simulink model "Porsche930Turbo_Model_V0"  (R2025b)
settings: Solver=ode3  StartTime=0.0  StopTime=1800  FixedStep=0.005  MaxStep=0.01  RelTol=1e-3
values from neighbouring files (symbols this model uses):
  a_front = (1 - CoG_front) * wb    (= 1.32912)    [Main.m]
  af = 1.77    [Main.m]
  bsfc = 395    [Main.m]
  cd = 0.39    [Main.m]
  crr = 0.015    [Main.m]
  distance_imola = s_track    [Main.m]
  eta_gb = 0.95    [Main.m]
  gear_numbers = [1, 2, 3, 4]    [Main.m]
  gear_ratios = [2.25, 1.30, 0.89, 0.625]    [Main.m]
  gear_shift_tbl = [1, 2, 3, 4]    [Main.m]
  grade_imola = grade_track    [Main.m]
  kt = 1.65    [Main.m]
  m_eq = mg + (J_wheels / rw^2) + (J_drivetrain * i_avg^2 / rw^2)    [Main.m]
  mg = mc + (mh * np) + mp_hybrid    (= 1492.5)    [Main.m]
  mu_road = 0.9    [Main.m]
  n_ice = 0:dn:nd    [Main.m]
  ne_em = 0:dn:nemax_em    [Main.m]
  nparallel = 2    [Main.m]
  nseries = 96    [Main.m]
  rho_fuel = 0.75    [Main.m]
  ro = 1.204    [Main.m]
  rt = 4.222    [Main.m]
  rw = (dw * 25.4 / 2 + wt * art / 100) * 1e-3    (= 0.31345)    [Main.m]
  t_ice = zeros(size(n_ice))    [Main.m]
  t_roma_san_basilio = [0 1 2 3 4 5 6 7 8 9 10 11 ... (522 elements, 522x1)]    [ECE_EUDC_Artemis_Bologna_Roma_WLTC_EE_bus.mat]
  tau_turbo = 0.6    [Main.m]
  te_em = zeros(size(ne_em))    [Main.m]
  te_em_peak = zeros(size(ne_em))    [Main.m]
  temax_em = 230    [Main.m]
  tmax_ice = 412    [Main.m]
  track_length = 4909    [Main.m]
  v_cutoff_bp = [0, 0.5, 1.4, 50]    [Main.m]
  v_cutoff_tbl = [0, 0,   1,   1 ]    [Main.m]
  v_ref_imola = v_track_ms    [Main.m]
  v_shift_bp = [0, 18, 33, 48]    [Main.m]
  v_shift_bp_EMODE = [0, 5, 22, 35]    [Main.m]
  vkm_roma_san_basilio = [28.8 30.9 32.4 34.2 35.3 35.6 34.8 33.8 32.2 30.5 29.1 27.9 ... (522 elements, 522x1)]    [ECE_EUDC_Artemis_Bologna_Roma_WLTC_EE_bus.mat]
  wb = 2.272    [Main.m]
undefined symbols (not defined in the file or in its folder): SoC_Per
libraries: simulink x58
(part 5 of 5)

== system Porsche930Turbo_Model_V0/E-MOTOR/EM_model_v47b/Motor_Model/blockD/idq_max_MTC-I0/iq_mtcMax/0ck1 ==
  i : Inport
  Abs1 : Abs  SaturateOnIntegerOverflow=off
  Constant3 : Constant  Value=0
  Manual Switch3 : ManualSwitch  CurrentSetting=0
  MinMax1 : MinMax  Function=max  Inputs=2
  o : Outport
  wires:
  i/1 -> MinMax1/1, Abs1/1
  Abs1/1 -> Manual Switch3/1
  Manual Switch3/1 -> o/1
  MinMax1/1 -> Manual Switch3/2
  Constant3/1 -> MinMax1/2

== matlab function Porsche930Turbo_Model_V0/ECU/Hybrid_Mode/MATLAB Function ==
  settings: updateMethod=DISCRETE  sampleTime=0.01
  data: t_req input; t_ICE output; t_em output; t_em_max input; SoC input
function [t_ICE, t_em] = Engine_sweetspot_operation(t_req, t_em_max, SoC)

    %ENFORCE UNIFORM DOUBLE PRECISION (Prevents Coder Type-Mismatch)
    t_req    = double(t_req);
    t_em_max = double(t_em_max);
    SoC      = double(SoC);

    t_sweetspot = 380.0;   % [Nm] Optimal BSFC operating point (3.3L Boxer Turbo)

    % AUTOMATIC SOC NORMALIZATION
    if SoC > 1.0
        soc_norm = SoC / 100.0;
    else
        soc_norm = SoC;
    end

    % HIGH-SOC REGENERATION / RECHARGE DERATING (90% -> 95%)
    % Protects battery cells against overvoltage (4.2V/cell) and lithium plating.
    if soc_norm <= 0.90
        regen_factor = 1.0;
    elseif soc_norm < 0.95
        regen_factor = (0.95 - soc_norm) / 0.05;
    else
        regen_factor = 0.0; % Above 95%: Zero recharge allowed (t_em >= 0)
    end

    % HYSTERESIS RECOVERY STATE (20% -> 50%)
    persistent force_recharge;
    if isempty(force_recharge)
        force_recharge = false;
    end

    % Latch forced recharge below 20%, maintain until 50% is recovered
    if (soc_norm <= 0.20)
        force_recharge = true;
    elseif (soc_norm >= 0.50)
        force_recharge = false;
    end

    %TORQUE DISPATCHING (CONTINUOUS LAWS)
    if force_recharge
        %STATE A: FORCED BATTERY RECOVERY MODE
        if t_req <= 0.0
            % Deceleration / Braking: regenerative braking scaled by regen_factor
            t_ICE = 0.0;
            t_em  = regen_factor * max(t_req, -t_em_max);

        else
            % Smooth throttle tip-in charging ramp (0 to 80 Nm)
            % Eliminates the instant 230 Nm (45 kW) step jump on pedal touch
            k_ramp    = min(1.0, t_req / 80.0);
            t_gen_max = regen_factor * min(t_em_max, max(0.0, t_sweetspot - t_req));
            t_gen     = k_ramp * t_gen_max;

            t_ICE = t_req + t_gen;
            t_em  = -t_gen;
        end

    else
        % STATE B: NORMAL HYBRID MODE
        t_ev_max   = 90.0;    % [Nm] Pure EV threshold
        t_ice_full = 125.0;   % [Nm] Full sweet-spot threshold

        if t_req <= 0.0
            % Deceleration / Braking: scaled regenerative braking
            t_ICE = 0.0;
            t_em  = regen_factor * max(t_req, -t_em_max);

        elseif t_req <= t_ev_max
            % Low load: Pure Electric Vehicle (EV) mode
            t_ICE = 0.0;
            t_em  = t_req;

        elseif t_req < t_ice_full
            % Smooth linear blending zone (90 to 125 Nm)
            alpha          = (t_req - t_ev_max) / (t_ice_full - t_ev_max);
            t_charge_avail = regen_factor * t_em_max;
            t_target_ice   = min(t_sweetspot, t_req + t_charge_avail);
            
            t_ICE = alpha * t_target_ice;
            t_em  = t_req - t_ICE;

        elseif t_req <= t_sweetspot
            % Medium load: ICE sweet-spot charging modulated by regen_factor
            t_charge_avail = regen_factor * min(t_em_max, t_sweetspot - t_req);
            t_ICE = t_req + t_charge_avail;
            t_em  = -t_charge_avail;

        elseif t_req <= (t_sweetspot + t_em_max)
            % High load: ICE at 380 Nm + Electric Motor Boost assist
            t_ICE = t_sweetspot;
            t_em  = t_req - t_sweetspot;

        else
            % Peak load: Saturated electric boost + ICE
            t_em  = t_em_max;
            t_ICE = t_req - t_em;
        end
    end
end

== matlab function Porsche930Turbo_Model_V0/E-MOTOR/EM_model_v47b/Motor_Model/TF/ solver_TF ==
  data: a input; id output; iq output; discr output; r input; r1 input; b input; t input; theta input
function [id, iq, discr] = SolQuart_tf(a, r, r1, b, t, theta)
% [id, iq, discr] = SolQuart_tf(a, r, r1, b, t, theta)
% page 77 tesi liscio (torque follower with Ferrari's method)

thp2 = theta^2;
th1  = 1/thp2+1;
if r==1  %isomachine
    det = a^2-th1*(th1*t^2/a^2+2*t/theta+a^2-b^2);
    if det>=0
        id    = (-a+sqrt(det)) /th1;
        iq    = t/a;
        discr = 1;
    else
        id    = 0;
        iq    = 0;
        discr = 0;
    end
else    %every other case other than isomachine
    %r1 = 1-1/r;
    %risoluzione della quartica
    A1 = r^2*r1^2+r1^2/thp2;
    B1 = 2*a*r1^2*r^2+r^2*2*a*r1+2*a*r1/thp2;
    C1 = -2*t*r1/theta+2*r*t*r1/theta+a^2*r^2+a^2/thp2+r^2*a^2*r1^2+4*a^2*r^2*r1-b^2*r1^2;
    D1 = -2*t*a/theta+2*a*r*t/theta+2*a*r*t*r1/theta+2*a^3*r^2+2*r^2*a^3*r1-2*a*r1*b^2;
    E1 = th1*t^2+2*a^2*r*t/theta+r^2*a^4-b^2*a^2;

    A = B1/A1;
    B = C1/A1;
    C = D1/A1;
    D = E1/A1;

    Pr = A*C - 4*D - (B^2/3);
    Qr = 4*B*D -A^2*D - C^2+ B*(A*C-4*D)/3 - 2*(B^3/27);

    DeltaR = (Qr^2/4) + (Pr^3/27);
    
    if DeltaR>0 %studio il discriminante per vedere se è correlato alla id_TF
        Sdelt = sqrt(DeltaR);
        temp1 = -Qr/2+Sdelt;
        temp2 = -Qr/2-Sdelt;
        Ur  = sign(temp1) * (abs(temp1))^(1/3);
        Vr  = sign(temp2) * (abs(temp2))^(1/3);
        S1r = Ur+Vr+B/3;
    else
        thetag = atan(sqrt(-DeltaR)/(-Qr/2));
        if thetag<0
            thetag = thetag+pi;
        end
        S1r = 2*sqrt(-Pr/3)*cos((thetag)/3)+B/3;
    end
    
    temp1 = sqrt((A^2/4)-B+S1r);
    temp2 = (-C+A*S1r/2) / (2*(A^2/4-B+S1r));
    %soluzioni quartica (utili)(valide solo se discr>0)
    
    if r<1
        I   = (A/2)   + temp1;
        L   = (S1r/2) + temp1 * temp2;
        det = I^2-4*L;
        if det<0
            id = 0;
        else
            id = 0.5* (-I + sqrt(det));
        end
    else
        G   = (A/2)   - temp1;
        H   = (S1r/2) - temp1 * temp2;
        det = G^2-4*H;
        if det<0
            id = 0;
        else
            id = 0.5* (-G + sqrt(det));
        end
    end
    
    if id==0
        iq    = 0;
        discr = 0;
    else
        iq    = t/(a+r1*id);
        discr = 1;
    end
end

end %fcn end

== matlab function Porsche930Turbo_Model_V0/E-MOTOR/EM_model_v47b/Motor_Model/blockD/idq_max_MTV-I0/intersections_neg ==
  data: a input; id output; iq output; discr output; r input; b input; I0 input; theta input; t input
function[id, iq, discr] = SolQuart_tfrs(a, r, b, I0, theta, t)
% [id, iq, discr] = SolQuart_tfrs(a, r, b, I0, theta, t)

thp2 = theta^2;
th1  = 1/thp2+1;
if r==1   %isomachine
    At  = (+I0^2*th1*thp2/a+thp2*a-thp2*b^2/a);
    Bt  = -I0^2+I0^4*th1^2*thp2/4/a^2+a^2*thp2/4+b^4*thp2/4/a^2+I0^2*...
          th1*thp2/2-I0^2*th1*thp2/a^2*b^2/2-thp2*b^2/2;
    det = At^2-4*(1+thp2)*Bt;
    if det>=0
        if t>=0
            id = (-At -sqrt(det)) / (2*(1+thp2));
        else
            id = (-At +sqrt(det)) / (2*(1+thp2));
        end
        iq   = -I0^2*th1*theta/(2*a)-id*theta-a*theta/2+b^2*theta/(2*a);
        discr = 0;
    else
        id    = 1000;
        iq    = 0;
        discr = 1;
    end

else      %every other case other than isomachine
    % risoluzione quartica (a,b,c,d a pag. 75, eq 3.31 )
    A1 = -4/thp2-4*r^2/thp2+8*r/thp2-th1^2-r^4-1/theta^4+2*th1*r^2+2*th1/thp2-2*r^2/thp2;
    B1 = 8*a*r/thp2-8*a*r^2/thp2+4*th1*a*r^2-4*r^4*a-4/thp2*a*r^2;
    C1 = 4/thp2*I0^2+4*r^2/thp2*I0^2-8*r/thp2*I0^2- 4*a^2*r^2/thp2+2*...
         th1^2*I0^2-4*a^2*r^4-2*b^2*th1+2*b^2*r^2+2*b^2/thp2+2*th1*a^2*r^2-2*...
         th1*I0^2*r^2-2*th1*I0^2/thp2-2*a^2*r^2/thp2-2*a^2*r^4;
    D1 = -8*a*r/thp2*I0^2+8*a*r^2*I0^2/thp2+4*b^2*a*r^2-4*I0^2*th1*a*r^2-4*a^3*r^4;
    E1 = 4*a^2*r^2*I0^2/thp2-b^4-th1^2*I0^4-a^4*r^4+2*b^2*th1*I0^2+2*b^2*a^2*r^2-2*I0^2*a^2*r^2*th1;

    A = B1/A1;
    B = C1/A1;
    C = D1/A1;
    D = E1/A1;
    
    Pr = A*C - 4*D - (B^2/3);
    Qr = 4*B*D - A^2*D - C^2 + B*(A*C-4*D)/3 - 2*(B^3/27);
    
    DeltaR = (Qr^2/4) + (Pr^3/27);
    
    if DeltaR>=0 
        %(se il discriminante è >0, allora il radicando è reale. Facendo la radice
        %cubica si ottiene una soluzione reale e 2 immaginarie. Le immaginarie
        %si ottengono moltiplicando la reale per (-1/2 +- irad3/2).
        Sdelt = sqrt(DeltaR);
        temp1 = -Qr/2+Sdelt;
        temp2 = -Qr/2-Sdelt;
        Ur  = sign(temp1) * (abs(temp1))^(1/3);
        Vr  = sign(temp2) * (abs(temp2))^(1/3);
        S1r = Ur+Vr+B./3;
    else
        thetag = atan(sqrt(-DeltaR)/(-Qr/2));
        if thetag<0
            thetag = thetag+pi;
        end
        S1r = 2*sqrt(-Pr/3)*cos((thetag)/3)+B/3;
    end
    
    det   = (A^2/4)-B+S1r;
    if det>=0
        temp1 = sqrt(det);
        temp2 = (-C+A*S1r/2) / (2*(A^2/4-B+S1r));
        %calcolo soluzioni quartica utili
        
        if r > 1
            G   = (A/2)   - temp1;
            H   = (S1r/2) - temp1 * temp2;
            det = G^2-4*H;
            if det<0
                id    = 0;
                discr = 1;
            else
                discr = 0;
                if t>=0
                    id = 0.5* (-G -sqrt(det));
                else
                    id = 0.5* (-G +sqrt(det));
                end
            end
        else 
            I   = (A/2)   + temp1;
            L   = (S1r/2) + temp1 * temp2;
            det = I^2-4*L;
            if det<0
                id    = 0;
                discr = 1;
            else
                discr = 0;
                if t>=0
                    id  = 0.5* (-I -sqrt(det));
                else
                    id  = 0.5* (-I +sqrt(det));
                end
            end
        end

        if discr==1
            iq    = 0;
            discr = 1;
        else
            iq_t = I0^2-id^2;
            if (iq_t<0 && r<=1)
                id   = 0;
                iq_t = 0;
            end
            if r<=1
                B   = (2*a*r/theta-2*id/theta+2*id*r/theta);
                C   = -b^2+r^2*a^2+id^2*r^2+id^2/thp2+2*a*id*r^2;
                det = B^2-4*C*th1;
                if det>=0
                    discr = 0;
                    if t>=0
                        iq = (-B +sqrt(det)) /(2*th1);
                    else
                        iq = -sqrt(iq_t);
                    end
                else
                    iq    = 0;
                    discr = 1;
                end
            else
                discr = 0;
                if t>=0
                    iq =  sqrt(iq_t);
                else
                    iq = -sqrt(iq_t);
                end
            end
        end
    else
        id    = 0;
        iq    = 0;
        discr = 1;
    end

end

end % end fcn

== matlab function Porsche930Turbo_Model_V0/E-MOTOR/EM_model_v47b/Motor_Model/blockD/idq_max_MTV-I0/intersections_pos ==
  data: a input; id output; iq output; discr output; r input; b input; I0 input; theta input; t input
function[id, iq, discr] = SolQuart_tfrs(a, r, b, I0, theta, t)
% [id, iq, discr] = SolQuart_tfrs(a, r, b, I0, theta, t)

thp2 = theta^2;
th1  = 1/thp2+1;
if r==1    %isomachine
    At  = +I0^2*th1*thp2/a + thp2*a - thp2*b^2/a;
    Bt  = -I0^2 + I0^4*th1^2*thp2/4/a^2 + a^2*thp2/4 + b^4*thp2/4/a^2 + ...
           I0^2*th1*thp2/2 - I0^2*th1*thp2/a^2*b^2/2 - thp2*b^2/2;
    det = At^2-4*(1+thp2)*Bt;
    if det>=0
        if t>=0
            id = (-At -sqrt(det)) / (2*(1+thp2));
        else
            id = (-At +sqrt(det)) / (2*(1+thp2));
        end
        iq   = -I0^2*th1*theta/(2*a)-id*theta-a*theta/2+b^2*theta/(2*a);
        discr = 0;
    else
        id    = 1000;
        iq    = 0;
        discr = 1;
    end

else     %every other case other than isomachine
    % risoluzione quartica (a,b,c,d a pag. 75, eq 3.31 )
    A1 = -4/thp2-4*r^2/thp2+8*r/thp2-th1^2-r^4-1/theta^4+2*th1*r^2+2*th1/thp2-2*r^2/thp2;
    B1 = 8*a*r/thp2-8*a*r^2/thp2+4*th1*a*r^2-4*r^4*a-4/thp2*a*r^2;
    C1 = 4/thp2*I0^2+4*r^2/thp2*I0^2-8*r/thp2*I0^2- 4*a^2*r^2/thp2 + ...
         2*th1^2*I0^2-4*a^2*r^4-2*b^2*th1+2*b^2*r^2+2*b^2/thp2+2*th1*a^2*r^2 - ...
         2*th1*I0^2*r^2-2*th1*I0^2/thp2-2*a^2*r^2/thp2-2*a^2*r^4;
    D1 = -8*a*r/thp2*I0^2+8*a*r^2*I0^2/thp2+4*b^2*a*r^2-4*I0^2*th1*a*r^2-4*a^3*r^4;
    E1 = 4*a^2*r^2*I0^2/thp2-b^4-th1^2*I0^4-a^4*r^4+2*b^2*th1*I0^2+2*b^2*a^2*r^2-2*I0^2*a^2*r^2*th1;

    A = B1/A1;
    B = C1/A1;
    C = D1/A1;
    D = E1/A1;
    
    Pr = A*C - 4*D - (B^2/3);
    Qr = 4*B*D - A^2*D - C^2 + B*(A*C-4*D)/3 - 2*(B^3/27);
    
    DeltaR = (Qr^2/4) + (Pr^3/27);
    
    if DeltaR>=0 
        %(se il discriminante è >0, allora il radicando è reale. Facendo la radice
        %cubica si ottiene una soluzione reale e 2 immaginarie. Le immaginarie
        %si ottengono moltiplicando la reale per (-1/2 +- irad3/2).
        Sdelt = sqrt(DeltaR);
        temp1 = -Qr/2+Sdelt;
        temp2 = -Qr/2-Sdelt;
        Ur  = sign(temp1) * (abs(temp1))^(1/3);
        Vr  = sign(temp2) * (abs(temp2))^(1/3);
        S1r = Ur+Vr+B./3;
    else
        thetag = atan(sqrt(-DeltaR)/(-Qr/2));
        if thetag<0
            thetag = thetag+pi;
        end
        S1r = 2*sqrt(-Pr/3)*cos((thetag)/3)+B/3;
    end
    
    det = (A^2/4)-B+S1r;
    if det>=0
        temp1 = sqrt(det);
        temp2 = (-C+A*S1r/2) / (2*(A^2/4-B+S1r));
        %calcolo soluzioni quartica utili
        
        if r > 1
            G   = (A/2)   - temp1;
            H   = (S1r/2) - temp1 * temp2;
            det = G^2-4*H;
            if det<0
                id    = 0;
                discr = 1;
            else
                discr = 0;
                if t>=0
                    id = 0.5* (-G -sqrt(det));
                else
                    id = 0.5* (-G +sqrt(det));
                end
            end
        else 
            I   = (A/2)   + temp1;
            L   = (S1r/2) + temp1 * temp2;
            det = I^2-4*L;
            if det<0
                id    = 0;
                discr = 1;
            else
                discr = 0;
                if t>=0
                    id  = 0.5* (-I -sqrt(det));
                else
                    id  = 0.5* (-I +sqrt(det));
                end
            end
        end

        if discr==1
            iq    = 0;
            discr = 1;
        else
            iq_t = I0^2-id^2;
            if (iq_t<0 && r<=1)
                id   = 0;
                iq_t = 0;
            end
            if r<=1
                B   = (2*a*r/theta-2*id/theta+2*id*r/theta);
                C   = -b^2+r^2*a^2+id^2*r^2+id^2/thp2+2*a*id*r^2;
                det = B^2-4*C*th1;
                if det>=0
                    discr = 0;
                    if t>=0
                        iq = (-B +sqrt(det)) /(2*th1);
                    else
                        iq = -sqrt(iq_t);
                    end
                else
                    iq    = 0;
                    discr = 1;
                end
            else
                discr = 0;
                if t>=0
                    iq =  sqrt(iq_t);
                else
                    iq = -sqrt(iq_t);
                end
            end
        end
    else
        id    = 0;
        iq    = 0;
        discr = 1;
    end

end

end % end fcn

== matlab function Porsche930Turbo_Model_V0/E-MOTOR/EM_model_v47b/Motor_Model/MTV/solver_MTV_neg ==
  data: a input; id output; r input; r1 input; b input; theta input; iq output; t input
function [id, iq] = SolQuart_mtv(a, r, r1, b, theta, t)
% [id, iq] = SolQuart_mtv(a, r, r1, b, theta, t)
% page 77 tesi liscio (Ferrari's method)

thp2 = theta^2;
th1  = 1/thp2+1;
if r==1   %isomachine
    
    id    = -a*thp2/(thp2+1);
    if t>0 
        iq = (-2*a/theta + sqrt((2*a/theta)^2-4*th1*(id^2*th1+2*id*a+a^2-b^2))) / (2*th1);
    else
        iq = (-2*a/theta - sqrt((2*a/theta)^2-4*th1*(id^2*th1+2*id*a+a^2-b^2))) / (2*th1);
    end
    
else   %every other case other than isomachine
    %r1 = 1-1/r;

    C2 = (a*r^2+a/thp2+a*r^2*r1) /(r1*th1);
    D2 = (r1*r^2+r1/thp2)        /(r1*th1);
    E2 = (a^2*r^2)               /(th1*r1);

    %risoluzione della quartica
    A1 = (4*D2/thp2+4*D2/thp2*r^2-8*r*D2/thp2-th1^2*D2^2-r^4-1/theta^4-...
         2*th1*D2*r^2-2*th1*D2/thp2-2*r^2/thp2);
    B1 = (4*C2/thp2+4*r^2*C2/thp2-8*r*C2/thp2-8*a*r*D2/thp2+8*a*r^2*D2/thp2-2*...
         th1^2*C2*D2-2*th1*C2*r^2-2*th1*C2/thp2-4*th1*D2*a*r^2-4*r^4*a-4*a*r^2/thp2);
    C1 = (-8*a*r*C2/thp2+8*a*r^2*C2/thp2+4*a^2*r^2*D2/thp2+4*E2/thp2+4*r^2*...
         E2/thp2-8*r*E2/thp2-th1^2*C2^2-4*a^2*r^4+2*b^2*th1*D2+2*b^2*r^2+2*...
         b^2/thp2-4*th1*C2*a*r^2-2*th1^2*D2*E2-2*th1*D2*r^2*a^2-2*th1*E2*r^2-2*...
         th1*E2/thp2-2*r^4*a^2-2*r^2*a^2/thp2);
    D1 = (-8*a*r*E2/thp2+8*a*r^2*E2/thp2+4*a^2*r^2*C2/thp2+2*b^2*th1*C2+4*...
         b^2*a*r^2-2*th1^2*C2*E2-2*th1*C2*r^2*a^2-4*th1*E2*a*r^2-4*r^4*a^3);
    E1 = 4*a^2*r^2*E2/thp2-b^4-th1^2*E2^2-r^4*a^4+2*b^2*th1*E2+2*b^2*r^2*a^2-2*th1*E2*r^2*a^2;

    A = B1/A1;
    B = C1/A1;
    C = D1/A1;
    D = E1/A1;

    Pr = A*C - 4*D - (B^2/3);
    Qr = 4*B*D - A^2*D - C^2+ B*(A*C-4*D)/3 + 2* ((-B)^3/27);

    DeltaR = (Qr^2/4) + (Pr^3/27);
    
    if DeltaR>0 %studio il discriminante per vedere se è correlato alla id
        Sdelt = sqrt(DeltaR);
        temp1 = -Qr/2+Sdelt;
        temp2 = -Qr/2-Sdelt;
        Ur  = sign(temp1) * (abs(temp1))^(1/3);
        Vr  = sign(temp2) * (abs(temp2))^(1/3);
        S1r = Ur+Vr+B/3;
    else
        thetag = atan(sqrt(-DeltaR)/(-Qr/2));
        if thetag<0
            thetag = thetag+pi;
        end
        S1r = 2*sqrt(-Pr/3)*cos(thetag./3)+B/3;
    end
    
    temp1 = sqrt((A^2/4)-B+S1r);
    temp2 = (-C+A*S1r/2) / (2*(A^2/4-B+S1r));
    %soluzioni quartica (utili) (valide solo se discr>0)
    
    if r<1
        I   = (A/2)   + temp1;
        L   = (S1r/2) + temp1 * temp2;
        det = I^2-4*L;
        if det<0
            id  = 0;
        else
            if t>0
                id  = 0.5* (-I +sqrt(det));
            else
                id  = 0.5* (-I -sqrt(det));
            end
        end
    else
        G   = (A/2)   - temp1;
        H   = (S1r/2) - temp1 * temp2;
        det = G^2-4*H;
        if det<0
            id  = 0;
        else
            if t>0
                id  = 0.5* (-G -sqrt(det));
            else
                id  = 0.5* (-G +sqrt(det));
            end
        end
    end
    
    if id==0
        iq = 0;
    else 
        if  (C2*id+D2*id^2+E2)>0
            B3 = (2*a*r/theta-2*id/theta+2*id*r/theta);
            C3 = -b^2+r^2*a^2+id^2*r^2+id^2/thp2+2*a*id*r^2;
            if t>=0
                iq = (-B3+sqrt(B3^2-4*C3*th1)) /(2*th1);
            else
                iq = (-B3-sqrt(B3^2-4*C3*th1)) /(2*th1);
            end
        else
            iq = 0;
        end
    end
    
end

end %fcn end

== matlab function Porsche930Turbo_Model_V0/E-MOTOR/EM_model_v47b/Motor_Model/MTC/ solver_MTC ==
  data: a input; id output; iq output; discr output; r input; r1 input; t input
function[id, iq, discr] = SolQuart_mtc(a, r, r1, t)
% [id, iq, discr] = SolQuart_mtc(a, r, r1, t)

if r==1    %isomachine
    id    = 0;
    iq    = t/a;
    discr = 1;
else       %every other case other than isomachine
    % risoluzione quartica (a,b,c,d a pag. 75, eq 3.31 )
    %r1   = 1-1/r;
    r1p3 = r1^3;
    A = (3*a*r1^2) /r1p3;
    B = (3*a^2*r1) /r1p3;
    C = (a^3)      /r1p3;
    D = -(t^2*r1)  /r1p3;
    
    Pr = A*C - 4*D - (B^2/3);
    Qr = 4*B*D - A^2*D - C^2 + B*(A*C-4*D)/3 - 2*(B^3/27);
    
    DeltaR = (Qr^2/4)+(Pr^3/27);
    
    if DeltaR>=0
        discr = 1;
        %(se il discriminante è >0, allora il radicando è reale. Facendo la radice
        %cubica si ottiene una soluzione reale e 2 immaginarie. Le immaginarie
        %si ottengono moltiplicando la reale per (-1/2 +- irad3/2).
        Sdelt = sqrt(DeltaR);
        temp1 = -Qr/2 + Sdelt;
        temp2 = -Qr/2 - Sdelt;
        Ur  = sign(temp1) * (abs(temp1))^(1/3);
        Vr  = sign(temp2) * (abs(temp2))^(1/3);
        S1r = Ur+Vr+B./3;
        
        temp1 = sqrt((A^2/4)-B+S1r);
        temp2 = (-C+A*S1r/2) / (2*((A^2/4)-B+S1r));
        %calcolo soluzioni quartica utili
        
        if a==0
            if r>1.01
                id =  ((t^2*r1)/(r1p3))^(1/4);
            elseif r<0.99
                id = -((t^2*r1)/(r1p3))^(1/4);
            else
                id = 0;
            end
        else
            if r>1.01
                G  = (A/2)   - temp1;
                H  = (S1r/2) - temp1 * temp2;
                id = 0.5* (-G + sqrt(G^2-4*H));
            elseif r<0.99
                I  = (A/2)   + temp1;
                L  = (S1r/2) + temp1 * temp2;
                id = 0.5* (-I - sqrt(I^2-4*L));
            else
                id = 0;
            end
        end

        if t>0
            d  =  id^2 + a*id/r1;
            iq =  sqrt(max(0,d));
        else
            d  =  id^2 + a*id/r1;
            iq = -sqrt(max(0,d));
        end

    else
        id    = 0;
        iq    = 0;
        discr = 0;
    end
end
   
end % fcn end

== stateflow chart Porsche930Turbo_Model_V0/Battery Pack/Subsystem/BMS/Chart ==
  state NormalState
    en:
    StopConditionOut = false;
    CurrentCondition = false;
  state Fault
    en:
    StopConditionOut = false;
    CurrentCondition = true;
    k = 0;
    during:
    k = k + 1;
    if k == 1000
    StopConditionOut = true;
    end
  (default) -> NormalState
  NormalState -> Fault : [StopCondition == 1]
  data: StopCondition input boolean; StopConditionOut output boolean; k local single; CurrentCondition output boolean

== matlab function Porsche930Turbo_Model_V0/E-MOTOR/EM_model_v47b/Motor_Model/MTV/solver_MTV_pos ==
  data: a input; id output; r input; r1 input; b input; theta input; iq output; t input
function [id, iq] = SolQuart_mtv(a, r, r1, b, theta, t)
% [id, iq] = SolQuart_mtv(a, r, r1, b, theta, t)
% page 77 tesi liscio (Ferrari's method)

thp2 = theta^2;
th1  = 1/thp2+1;
if r==1 % isomachine
    
    id    = -a*thp2/(thp2+1);
    if t>0 
        iq = (-2*a/theta + sqrt((2*a/theta)^2-4*th1*(id^2*th1+2*id*a+a^2-b^2))) / (2*th1);
    else
        iq = (-2*a/theta - sqrt((2*a/theta)^2-4*th1*(id^2*th1+2*id*a+a^2-b^2))) / (2*th1);
    end
    
else   %every other case other than isomachine
    %r1 = 1-1/r;

    C2 = (a*r^2+a/thp2+a*r^2*r1) /(r1*th1);
    D2 = (r1*r^2+r1/thp2)        /(r1*th1);
    E2 = (a^2*r^2)               /(th1*r1);

    %risoluzione della quartica
    A1 = (4*D2/thp2+4*D2/thp2*r^2-8*r*D2/thp2-th1^2*D2^2-r^4-1/theta^4-...
         2*th1*D2*r^2-2*th1*D2/thp2-2*r^2/thp2);
    B1 = (4*C2/thp2+4*r^2*C2/thp2-8*r*C2/thp2-8*a*r*D2/thp2+8*a*r^2*D2/thp2-2*...
         th1^2*C2*D2-2*th1*C2*r^2-2*th1*C2/thp2-4*th1*D2*a*r^2-4*r^4*a-4*a*r^2/thp2);
    C1 = (-8*a*r*C2/thp2+8*a*r^2*C2/thp2+4*a^2*r^2*D2/thp2+4*E2/thp2+4*r^2*...
         E2/thp2-8*r*E2/thp2-th1^2*C2^2-4*a^2*r^4+2*b^2*th1*D2+2*b^2*r^2+2*...
         b^2/thp2-4*th1*C2*a*r^2-2*th1^2*D2*E2-2*th1*D2*r^2*a^2-2*th1*E2*r^2-2*...
         th1*E2/thp2-2*r^4*a^2-2*r^2*a^2/thp2);
    D1 = (-8*a*r*E2/thp2+8*a*r^2*E2/thp2+4*a^2*r^2*C2/thp2+2*b^2*th1*C2+4*...
         b^2*a*r^2-2*th1^2*C2*E2-2*th1*C2*r^2*a^2-4*th1*E2*a*r^2-4*r^4*a^3);
    E1 = 4*a^2*r^2*E2/thp2-b^4-th1^2*E2^2-r^4*a^4+2*b^2*th1*E2+2*b^2*r^2*a^2-2*th1*E2*r^2*a^2;

    A = B1/A1;
    B = C1/A1;
    C = D1/A1;
    D = E1/A1;

    Pr = A*C - 4*D - (B^2/3);
    Qr = 4*B*D - A^2*D - C^2+ B*(A*C-4*D)/3 - 2*(B^3/27);

    DeltaR = (Qr^2/4) + (Pr^3/27);
    
    if DeltaR>0 %studio il discriminante per vedere se è correlato alla id
        Sdelt = sqrt(DeltaR);
        temp1 = -Qr/2+Sdelt;
        temp2 = -Qr/2-Sdelt;
        Ur  = sign(temp1) * (abs(temp1))^(1/3);
        Vr  = sign(temp2) * (abs(temp2))^(1/3);
        S1r = Ur+Vr+B/3;
    else
        thetag = atan(sqrt(-DeltaR)/(-Qr/2));
        if thetag<0
            thetag = thetag+pi;
        end
        S1r = 2*sqrt(-Pr/3)*cos(thetag./3)+B/3;
    end
    
    temp1 = sqrt((A^2/4)-B+S1r);
    temp2 = (-C+A*S1r/2) / (2*(A^2/4-B+S1r));
    %soluzioni quartica (utili) (valide solo se discr>0)
    
    if r<1
        I   = (A/2)   + temp1;
        L   = (S1r/2) + temp1 * temp2;
        det = I^2-4*L;
        if det<0
            id  = 0;
        else
            if t>=0
                id  = 0.5* (-I +sqrt(det));
            else
                id  = 0.5* (-I -sqrt(det));
            end
        end
    else
        G   = (A/2)   - temp1;
        H   = (S1r/2) - temp1 * temp2;
        det = G^2-4*H;
        if det<0
            id  = 0;
        else
            if t>0
                id  = 0.5* (-G -sqrt(det));
            else
                id  = 0.5* (-G +sqrt(det));
            end
        end
    end
    
    if id==0
        iq = 0;
    else 
        if  (C2*id+D2*id^2+E2)>0
            B3 = (2*a*r/theta-2*id/theta+2*id*r/theta);
            C3 = -b^2+r^2*a^2+id^2*r^2+id^2/thp2+2*a*id*r^2;
            if t>=0
                iq = (-B3 +sqrt(B3^2-4*C3*th1)) /(2*th1);
            else
                iq = (-B3 -sqrt(B3^2-4*C3*th1)) /(2*th1);
            end
        else
            iq = 0;
        end
    end
    
end

end %fcn end

== matlab function Porsche930Turbo_Model_V0/Battery Pack/Subsystem/Thermal Model/air cooling ==
  data: v_car input; Q_cool output; T_cell input; T_amb input
function Q_cool = air_cooling(v_car, T_cell, T_amb)
   
    v = double(v_car);
    Tc = double(T_cell);
    Ta = double(T_amb);

    % Parameters of heat exchange of air
    hA_passiv = 8.0;   % [W/K]
    hA_fan_max = 22.0;  % [W/K]
    k_ram_air  = 0.85;  % Air from front inlets [W/(K*(m/s))]

    if Tc > 38.0
        fan_cmd = 1.0;  
    elseif Tc > 32.0
        fan_cmd = 0.5;  
    else
        fan_cmd = 0.0; 
    end

    hA_eff = hA_passiv + (fan_cmd * hA_fan_max) + (k_ram_air * abs(v));

    % Heat exchanged
    if Tc > Ta
        Q_val = hA_eff * (Tc - Ta);
    else
        Q_val = 0.0;
    end

    Q_cool = cast(Q_val, 'like', T_cell);
end

== matlab function Porsche930Turbo_Model_V0/Lap TIme/MATLAB Function ==
  data: t input; lap_time_str output; dist input; L_track input; lap_time_sec output; is_finished output
function [lap_time_str, lap_time_sec, is_finished] = Lap_Timer_Logic(t, dist, L_track)
    % CRONOMETRO DIGITALE CIRCUITO DI IMOLA (MM:SS.mmm)
    persistent latched_time finished
    if isempty(latched_time)
        latched_time = 0.0;
        finished = false;
    end

    % Verifica se la Porsche ha tagliato il traguardo (4909 m)
    if dist >= L_track
        if ~finished
            latched_time = t;
            finished = true;
        end
        t_curr = latched_time;
        is_finished = true;
    else
        t_curr = t;
        is_finished = false;
    end

    lap_time_sec = t_curr;

    % Calcolo di Minuti, Secondi e Millesimi
    mins   = int32(floor(t_curr / 60));
    secs   = int32(floor(mod(t_curr, 60)));
    millis = int32(floor(mod(t_curr, 1) * 1000));

    % Formattazione stringa XX:XX:XXX
    lap_time_str = string(sprintf('%02d:%02d.%03d', mins, secs, millis));
end
